simulink model "Regelkreis_T4"  (R2025a)
settings: Solver=VariableStepAuto  StartTime=0.0  StopTime=60  RelTol=1e-3
model workspace (MAT data in the model file):
  K_I = 1
  T_1 = [1 1]
settings Model: Creator=ofm31594  LastModifiedBy=ofm31594

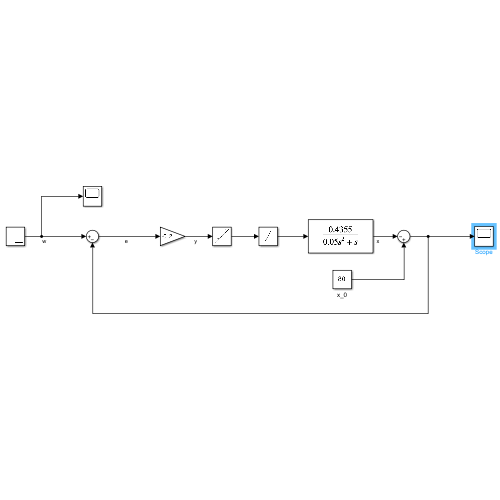
[thumbnail: Simulink's stored preview of the top-level diagram]
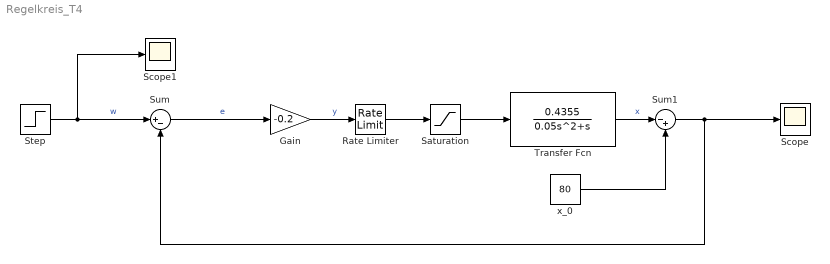
== system Regelkreis_T4 ==
  Gain : Gain  Gain=-0.2
  Rate Limiter : RateLimiter  RisingSlewLimit=0.04/0.02  FallingSlewLimit=-0.04/0.02  SampleTimeMode=inherited
  Saturation : Saturate  UpperLimit=100  LowerLimit=-100
  Scope : Scope
      settings: ActiveDisplayYMinimum=23.980468805242506  ActiveDisplayYMaximum=31.024648055905882
  Scope1 : Scope
      settings: ActiveDisplayYMinimum=-1  ActiveDisplayYMaximum=1
  Step : Step  Time=0.01  Before=80  After=25  SampleTime=0
  Sum : Sum  Inputs=|+-
  Sum1 : Sum  Inputs=|-+
  Transfer Fcn : TransferFcn  Numerator=0.4355  Denominator="[ 0.05 1  0]"
  x_0 : Constant  Value=80
  wires:
  Sum/1 -> Gain/1  "e"
  Gain/1 -> Rate Limiter/1  "y"
  Step/1 -> Scope1/1, Sum/1  "w"
  Sum1/1 -> Sum/2, Scope/1
  Transfer Fcn/1 -> Sum1/1  "x"
  x_0/1 -> Sum1/2
  Rate Limiter/1 -> Saturation/1
  Saturation/1 -> Transfer Fcn/1
